simulink model "BatteryEstim3RC_PTBS_EQ_v1"  (R2021b)
settings: Solver=VariableStepAuto  StartTime=0.0  StopTime=mp.t(end)  FixedStep=0.01  MaxStep=60  RelTol=1e-3
values from neighbouring files (symbols this model uses):
  mpg = mp    [test_experimentalData.m]
  Rx = [0.00360983119348 0.0168144449279 0.13578095254 0.00425221519399 0.0157895308187 0.0287753886048 0.0043185556022 0.0204140342686 0.066625855529 0.00438636985678 0.0198858505729 0.0147056919192 ... (144 elements, 3x48)]    [20230919_data_fit.mat]
  Tx = [1.35234061928 30.5436923263 327.790937158 1.33969974341 28.0604597727 433.455062576 1.34425640628 28.3500143142 439.319267322 1.25167719089 28.0276573618 175.175429763 ... (144 elements, 3x48)]    [20230919_data_fit.mat]
libraries: autolibrcnetworksystem x1, autolibbatterycommon x1
settings Model: ModifiedByFormat=The MathWorks, Inc.  Creator=The MathWorks, Inc.  LastModifiedBy=The MathWorks, Inc.
settings SolverCC: AlgebraicLoopSolver=TrustRegion
settings DataIOCC: ExternalInput=[mp.t, mp.i]  LoadExternalInput=on  DSMLogging=off  SaveTime=off  ReturnWorkspaceOutputs=off
settings DebuggingCC: SFMachineParentedDataDiag=warning  ArithmeticOperatorsInVariantConditions=warning
settings SFSimCC: SimUseLocalCustomCode=off  CustomCodeUndefinedFunction=UseInterfaceOnly
settings RTWCC: RTWUseLocalCustomCode=off
settings CodeAppCC: StateflowObjectComments=on

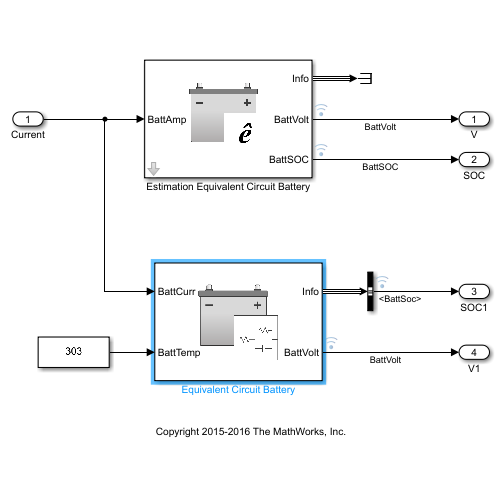
[thumbnail: Simulink's stored preview of the top-level diagram]
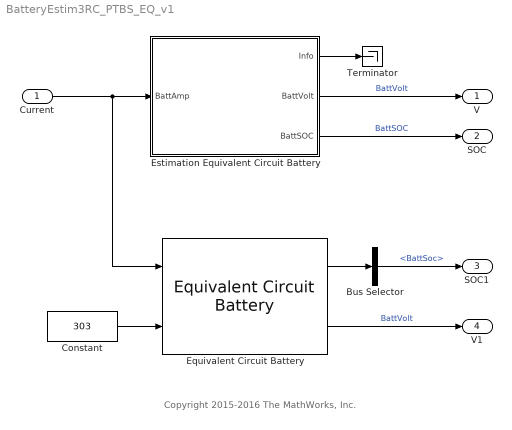
== system BatteryEstim3RC_PTBS_EQ_v1 ==
  note: Copyright 2015-2016 The MathWorks, Inc.
  Current : Inport
  Bus Selector : BusSelector  OutputSignals=BattSoc
  Constant : Constant  Value=303
  Equivalent Circuit Battery : autolibrcnetworksystem/Equivalent Circuit Battery  CapacityCtrl=Parameter  OutputVlt=Unfiltered  NumRC=3  Em=mpg.EmPrime  R0=mpg.R0Prime  SOC_BP=mpg.SOC_LUTPrime  Temperature_BP=mpg.TempPrime  BattCap=mpg.CapacityAhPrime  BattCapInit=mpg.CapacityAh - mpg.InitialChargeDeficitAh  InitialCapVoltage=mpg.InitialCapVoltage  Tc=1/1000  Vinit=4.193  R1=mpg.R1Prime  C1=mpg.C1Prime  R2=mpg.R2Prime  C2=mpg.C2Prime  R3=mpg.R3Prime  C3=mpg.C3Prime  R4=R4Prime  C4=C4Prime  R5=|  C5=|  Vu=Inf  Vl=-Inf  RefBlkName='autolibrcnetworksystem/Equivalent Circuit Battery'
      R5=|
      | [0.010342 0.0012244;
      | 0.0067316 0.0011396;
      | 0.0051156 0.0012661;
      | 0.0043447 0.0012265;
      | 0.0038826 0.0011163;
      | 0.0034226 0.0009968;
      | 0.003346 0.0011458;
      | 0.0033222 0.001345;
      | 0.0033201 0.0013091;
      | 0.0032886 0.0010986;
      | 0.0028114 0.0010309]
      C5=|
      | [2287.7 11897;
      | 6122 24515;
      | 18460 42098;
      | 20975 44453;
      | 15254 33098;
      | 10440 24492;
      | 13903 32975;
      | 16694 40007;
      | 15784 35937;
      | 12165 26430;
      | 9118 24795]
      settings: SourceProductBaseCode=PW
  Estimation Equivalent Circuit Battery : Subsystem  mask(Estimation Equivalent Circuit Battery){NumRC=3, Em=mpg.Em, R0=mpg.R0prime, SOC_BP=mpg.SOC_LUT, BattCap=mpg.CapacityAh, BattCapInit=mpg.CapacityAh - mpg.InitialChargeDeficitAh, InitialCapVoltage=mpg.InitialCapVoltage, R1=mpg.R1prime, C1=mpg.C1prime, R2=mpg.R2prime, C2=mpg.C2prime, R3=mpg.R3prime, C3=mpg.C3prime, R4=Rx(4,:), C4=Tx(4,:)./Rx(4,:), R5=[0.005 0.005 0.005 0.005 0.005 0.005], C5=[10000 10000 10000 10000 10000 10000], Vu=Inf, Vl=-Inf}
      mask prompts: NumRC "autoblks:autoblkParamEstRcBattery:blkPrm_NumRC"; Em "autoblks:autoblkParamEstRcBattery:blkPrm_Em"; R0 "autoblks:autoblkParamEstRcBattery:blkPrm_R0"; SOC_BP "autoblks:autoblkParamEstRcBattery:blkPrm_SOC_BP"; BattCap "autoblks:autoblkParamEstRcBattery:blkPrm_BattCap"; BattCapInit "autoblks:autoblkParamEstRcBattery:blkPrm_BattCapInit"; InitialCapVoltage "autoblks:autoblkParamEstRcBattery:blkPrm_InitialCapVoltage"; R1 "autoblks:autoblkParamEstRcBattery:blkPrm_R1"; C1 "autoblks:autoblkParamEstRcBattery:blkPrm_C1"; R2 "autoblks:autoblkParamEstRcBattery:blkPrm_R2"; C2 "autoblks:autoblkParamEstRcBattery:blkPrm_C2"; R3 "autoblks:autoblkParamEstRcBattery:blkPrm_R3"; C3 "autoblks:autoblkParamEstRcBattery:blkPrm_C3"; R4 "autoblks:autoblkParamEstRcBattery:blkPrm_R4"; C4 "autoblks:autoblkParamEstRcBattery:blkPrm_C4"; R5 "autoblks:autoblkParamEstRcBattery:blkPrm_R5"; C5 "autoblks:autoblkParamEstRcBattery:blkPrm_C5"; Vu "autoblks:autoblkParamEstRcBattery:blkPrm_Vu"; Vl "autoblks:autoblkParamEstRcBattery:blkPrm_Vl"
      mask help: autoblks:autoblkParamEstRcBattery:blkDesc
      mask init:
      | autoicon('pbbatteryparamest', gcb, 'Initialization');
      mask Help: eval('autoblkshelp(''pbbatteryrcnetworkpe'')');
      mask TypeOptions NumRC: autoblks:autoblkParamEstRcBattery:blkCmb_NumRC1 | autoblks:autoblkParamEstRcBattery:blkCmb_NumRC2 | autoblks:autoblkParamEstRcBattery:blkCmb_NumRC3 | autoblks:autoblkParamEstRcBattery:blkCmb_NumRC4 | autoblks:autoblkParamEstRcBattery:blkCmb_NumRC5
      mask Callback NumRC: autoicon('pbbatteryparamest', gcb, 'NumRCPopup');
      mask DialogControl Container9 Prompt: autoblks:autoblkParamEstRcBattery:blkDlg_Container9
      mask DialogControl NumRC Prompt: Number of series RC pairs:
      mask DialogControl Em Prompt: Open circuit voltage table data, Em [V]:
      mask DialogControl R0 Prompt: Series resistance table data, R0 [Ohm]:
      mask DialogControl SOC_BP Prompt: State of charge breakpoints, SOC_BP []:
      mask DialogControl BattCap Prompt: Battery capacity, BattCap [Ah]:
      mask DialogControl BattCapInit Prompt: Initial battery capacity, BattCapInit [Ah]:
      mask DialogControl InitialCapVoltage Prompt: Initial capacitor voltage, InitialCapVoltage [V]:
      mask DialogControl Container10 Prompt: autoblks:autoblkParamEstRcBattery:blkDlg_Container10
      mask DialogControl R1 Prompt: Network resistance table data, R1 [Ohm]:
      mask DialogControl C1 Prompt: Network capacitance table data, C1 [F]:
      mask DialogControl R2 Prompt: Network resistance table data, R2 [Ohm]:
      mask DialogControl C2 Prompt: Network capacitance table data, C2 [F]:
      mask DialogControl R3 Prompt: Network resistance table data, R3 [Ohm]:
      mask DialogControl C3 Prompt: Network capacitance table data, C3 [F]:
      mask DialogControl R4 Prompt: Network resistance table data, R4 [Ohm]:
      mask DialogControl C4 Prompt: Network capacitance table data, C4 [F]:
      mask DialogControl R5 Prompt: Network resistance table data, R5 [Ohm]:
      mask DialogControl C5 Prompt: Network capacitance table data, C5 [F]:
      mask DialogControl Container7 Prompt: autoblks:autoblkParamEstRcBattery:blkDlg_Container7
      mask DialogControl Vu Prompt: Upper Integrator Voltage Limit, Vu [V]:
      mask DialogControl Vl Prompt: Lower Integrator Voltage Limit, Vl [V]:
      mask Display:
      | IconInfo = autoicon('pbbatteryparamest', gcb, 'DrawCommands');
      | 
      | image(IconInfo.image, IconInfo.position);
      | 
      | for i = 1:numel(IconInfo.lconn)
      |     port_label('lconn', i, IconInfo.lconn{i})
      | end
      | 
      | for j = 1:numel(IconInfo.rconn)
      |     port_label('rconn', j, IconInfo.rconn{j})
      | end
      | 
      | for k = 1:numel(IconInfo.input)
      |     port_label('input', k, IconInfo.input{k})
      | end
      | 
      | for m = 1:numel(IconInfo.output)
      |     port_label('output', m, IconInfo.output{m})
      | end
  Terminator : Terminator
  V : Outport  VectorParamsAs1DForOutWhenUnconnected=off
  SOC : Outport  Port=2  VectorParamsAs1DForOutWhenUnconnected=off
  SOC1 : Outport  Port=3  VectorParamsAs1DForOutWhenUnconnected=off
  V1 : Outport  Port=4  VectorParamsAs1DForOutWhenUnconnected=off
  wires:
  Estimation Equivalent Circuit Battery/3(BattSOC) -> SOC/1  "BattSOC"
  Estimation Equivalent Circuit Battery/2(BattVolt) -> V/1  "BattVolt"
  Current/1 -> Equivalent Circuit Battery/1, Estimation Equivalent Circuit Battery/1(BattAmp)
  Estimation Equivalent Circuit Battery/1(Info) -> Terminator/1
  Equivalent Circuit Battery/1 -> Bus Selector/1
  Bus Selector/1 -> SOC1/1  "<BattSoc>"
  Equivalent Circuit Battery/2 -> V1/1  "BattVolt"
  Constant/1 -> Equivalent Circuit Battery/2

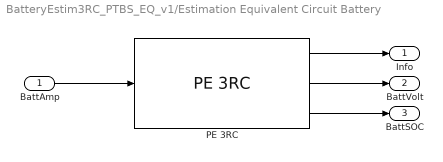
== system BatteryEstim3RC_PTBS_EQ_v1/Estimation Equivalent Circuit Battery ==
  BattAmp : Inport
  PE 3RC : autolibbatterycommon/PE 3RC  SystemSampleTime=-1  VariantControl=3  VariantActivationTime=update diagram  Latency=0  AutoFrameSizeCalculation=off
      settings: SourceProductBaseCode=PW
  Info : Outport  VectorParamsAs1DForOutWhenUnconnected=off
  BattVolt : Outport  Port=2  VectorParamsAs1DForOutWhenUnconnected=off
  BattSOC : Outport  Port=3  VectorParamsAs1DForOutWhenUnconnected=off
  wires:
  BattAmp/1 -> PE 3RC/1
  PE 3RC/3 -> BattSOC/1
  PE 3RC/2 -> BattVolt/1
  PE 3RC/1 -> Info/1
